simulink model "sheme"  (R2024a)
settings: Solver=VariableStepAuto  StartTime=0.0  StopTime=0.01  FixedStep=5e-6  MaxStep=5e-6  RelTol=1e-3
undefined symbols (not defined in the file or in its folder): den, num
settings Model: Creator=user  LastModifiedBy=user
settings SFSimCC: SimCustomHeaderCode="#include \"cheby1_filter.h\""  SimUserSources=cheby1_filter.c

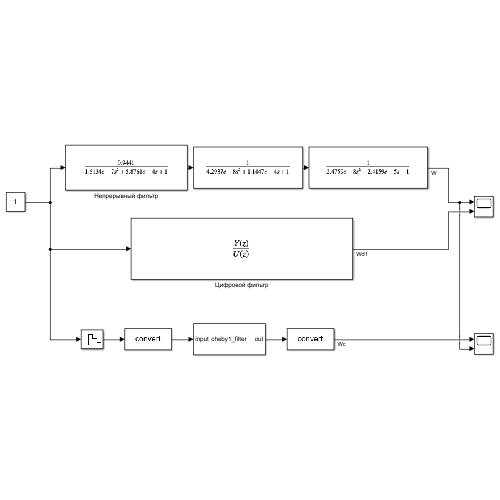
[thumbnail: Simulink's stored preview of the top-level diagram]
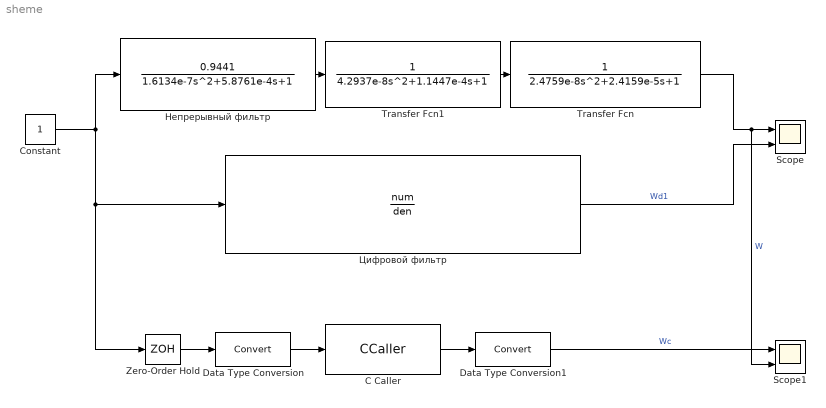
== system sheme ==
  C Caller : CCaller  FunctionName=cheby1_filter  PortSpecificationStruct="%)30     .    R ,   8    (     @         %    \"     (    !     0         %  0 \"0    $    _    07)G3F%M90  4&]R=$YA;64 4V-O<&4     26YD97@     5'EP90      4VEZ90      27-';&]B86P   X    P    !@    @    $          4    (     0    ,    !         !   P!O=70 #@   #     &    \"     0         !0    @    !     P    $         $  # &]U=  .    .     8    (    !          %    \"     $    &     0         0    !@   $]U='!U=   #@   #@    &    \"     8         !0    @    !     0    $         \"0    @               X    X    !@    @    $          4    (     0    8    !         !     &    <VEN9VQE   .    ,     8    (    !          %    \"     $    !     0         0  $ ,0    X    P    !@    @    ) @        4    (     0    $    !          (  0      #@   #@    &    \"     0         !0    @    !    !0    $         $     4   !I;G!U=     X    X    !@    @    $          4    (     0    4    !         !     %    :6YP=70    .    .     8    (    !          %    \"     $    %     0         0    !0   $EN<'5T    #@   #@    &    \"     8         !0    @    !     0    $         \"0    @               X    X    !@    @    $          4    (     0    8    !         !     &    <VEN9VQE   .    ,     8    (    !          %    \"     $    !     0         0  $ ,0    X    P    !@    @    ) @        4    (     0    $    !          (  0"  SampleTime=5e-5
  Constant : Constant
  Data Type Conversion : DataTypeConversion  SaturateOnIntegerOverflow=off  RndMeth=Floor
  Data Type Conversion1 : DataTypeConversion  SaturateOnIntegerOverflow=off  RndMeth=Floor
  Scope : Scope  NumInputPorts=2
  Scope1 : Scope  NumInputPorts=2
  Transfer Fcn : TransferFcn  Denominator=[2.4759e-8 2.4159e-5 1]
  Transfer Fcn1 : TransferFcn  Denominator=[4.2937e-8 1.1447e-4 1]
  Zero-Order Hold : ZeroOrderHold  SampleTime=5e-5
  Непрерывный фильтр : TransferFcn  Numerator=[0.9441]  Denominator=[1.6134e-7 5.8761e-4 1]
  Цифровой фильтр : DiscreteTransferFcn  Numerator=num  Denominator=den  SampleTime=5e-5
  wires:
  Непрерывный фильтр/1 -> Transfer Fcn1/1
  Transfer Fcn1/1 -> Transfer Fcn/1
  Цифровой фильтр/1 -> Scope/2  "Wd1"
  Transfer Fcn/1 -> Scope1/2, Scope/1  "W"
  Zero-Order Hold/1 -> Data Type Conversion/1
  Data Type Conversion/1 -> C Caller/1
  C Caller/1 -> Data Type Conversion1/1
  Constant/1 -> Zero-Order Hold/1, Цифровой фильтр/1, Непрерывный фильтр/1
  Data Type Conversion1/1 -> Scope1/1  "Wc"
